simulink model "Simple_1MW_EVSE_SC_Study"  (R2024b)
settings: Solver=FixedStepDiscrete  StartTime=0.0  StopTime=10.0  FixedStep=1e-4  RelTol=1e-3
undefined symbols (not defined in the file): DiscIntNeverNeededParam
libraries: spsCurrentMeasurementLib x3, spsSeriesRLCBranchLib x3, spsVoltageMeasurementLib x3, spsIdealSwitchLib x3, spsControlledCurrentSourceLib x1, spsControlledVoltageSourceLib x1, spsDCVoltageSourceLib x1, spspowerguiLib x1
settings Model: NumberOfSteps=10000  SnapshotInterval=10000  Creator=SUDHAK1  LastModifiedBy=SUDHAK1

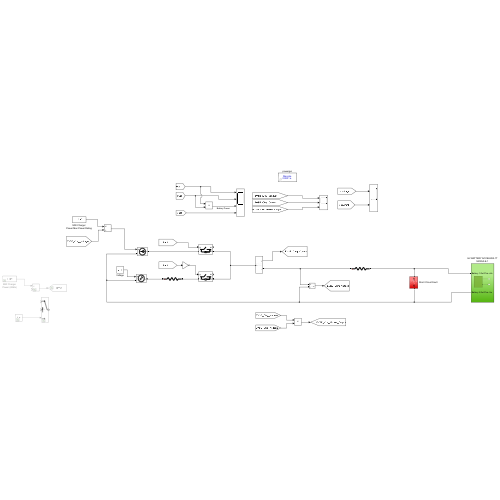
[thumbnail: Simulink's stored preview of the top-level diagram]
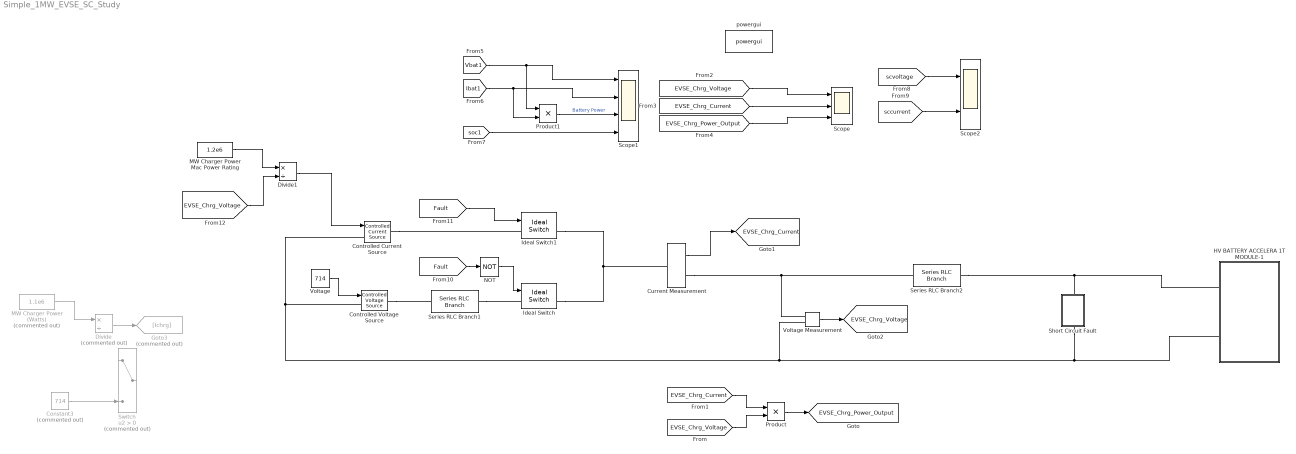
== system Simple_1MW_EVSE_SC_Study ==
  Constant3 : Constant  Commented=on  Value=714
  Controlled Current Source : spsControlledCurrentSourceLib/Controlled Current Source  Initialize=on  Source_Type=AC  Amplitude=0  Phase=0  Frequency=0  Measurements=None
  Controlled Voltage Source : spsControlledVoltageSourceLib/Controlled Voltage Source  Initialize=on  Source_Type=DC  Amplitude=0  Phase=0  Frequency=0  Measurements=None
  Current Measurement : spsCurrentMeasurementLib/Current Measurement  PhasorSimulation=off  OutputType=Complex  PSBequivalent=0
  Divide : Product  Commented=on  Inputs=*/
  Divide1 : Product  Inputs=*/
  Goto3 : Goto  Commented=on  GotoTag=Ichrg
  HV BATTERY ACCELERA 1T MODULE-1 : Subsystem
  Ideal Switch : spsIdealSwitchLib/Ideal Switch  Ron=1e-6  Lon=0  IC=0  Rs=1e5  Cs=inf  Measurements=on
  Ideal Switch1 : spsIdealSwitchLib/Ideal Switch  Ron=1e-6  Lon=0  IC=0  Rs=1e5  Cs=inf  Measurements=on
  MW Charger Power (Watts) : Constant  Commented=on  Value=1.1e6
  MW Charger Power Mac Power Rating : Constant  Value=1.2e6
  NOT : Logic  Operator=NOT  IconShape=distinctive  AllPortsSameDT=off  OutDataTypeStr=boolean
  Product : Product
  Product1 : Product
  Scope : Scope  NumInputPorts=3
  Scope1 : Scope  NumInputPorts=4
  Scope2 : Scope  NumInputPorts=2
  Series RLC Branch1 : spsSeriesRLCBranchLib/Series RLC Branch  LConnTagsString=__new0  RConnTagsString=__new0  BranchType=R  Resistance=(1000/1500)+0.3  Inductance=1e-3  SetiL0=off  InitialCurrent=0  Capacitance=1e-6  Setx0=off  InitialVoltage=0  Measurements=None
  Series RLC Branch2 : spsSeriesRLCBranchLib/Series RLC Branch  LConnTagsString=__new0  RConnTagsString=__new0  BranchType=R  Resistance=2e-3  Inductance=1e-3  SetiL0=off  InitialCurrent=0  Capacitance=1e-6  Setx0=off  InitialVoltage=0  Measurements=None
  Short Circuit Fault : Subsystem
      settings: PortSchema="{\"entries\":[{\"content\":{\"sides\":[{\"content\":{},\"type\":\"ConnectorPlacement.EquallySpacedRectSide\",\"uuid\":\"d1eece8f-50e0-4bd3-bd02-64a44f95c15f\"},{\"content\":{\"side\":\"RIGHT\"},\"type\":\"ConnectorPlacement.EquallySpacedRectSide\",\"uuid\":\"d3715762-f460-4a18-a379-b690b190937e\"},{\"content\":{\"connectorIds\":[\"LConn1\"],\"side\":\"TOP\"},\"type\":\"ConnectorPlacement.EquallySpacedRectSide\",\"uuid\":\"cdaaabb7-d644-4e36-8adb-959b7298db19\"},{\"content\":{\"connectorIds\":[\"RConn1\"],\"side\":\"BOTTOM\"},\"type\":\"ConnectorPlacement.EquallySpacedRectSide\",\"uuid\":\"a0244b95-e79a-4abc-836f-bd8cb9c3c8a7\"}]},\"type\":\"ConnectorPlacement.EquallySpacedConnector\",\"uuid\":\"f19808b0-397b-4bab-947c-d2711a911d87\"}],\"packageUris\":[\"http://schema.mathworks.com/mf0/Connector/R2020b\"],\"version\":\"1.0\"}"
  Switch : Switch  Commented=on  Criteria=u2 > Threshold  SaturateOnIntegerOverflow=off  InputSameDT=off
  Voltage : Constant  Value=714
  Voltage Measurement : spsVoltageMeasurementLib/Voltage Measurement  PhasorSimulation=off  OutputType=Complex  PSBequivalent=0
  powergui : spspowerguiLib/powergui  Priority=1  SimulationMode=Discrete  SampleTime=1e-4  frequency=60  Iterations=50  frequencyindice=0  Pbase=100e6  ErrMax=1e-4  UnitsV=kV  UnitsW=MW  buscounter=0  FunctionMessages=off  echomessages=off  EnableUseOfTLC=off  CurrentSourceSwitches=off  DisableSnubberDevices=off  DisableRonSwitches=off  DisableVfSwitches=off  DisplayEquations=off  AutomaticDiscreteSolvers=off  SolverType=Backward Euler  Interpol=off  ExternalGateDelay=off  methode=off  Ts=100  x0status=blocks  SPID=on  SwTol=0  HookPort=off  NonlinearTolerance=1e-4  nMaxIteration=100  ContinueOnMaxIteration=off  RestoreLinks=warning  ResistiveCurrentMeasurement=off  Frange=[0:2:500]  Ylog=off  Xlog=on  ShowGrid=off  save=off  variable=ZData  structure=0  ZoomFFT=off  StartTime=0.0  cycles=1  DisplayStyle=1  fundamental=60  FreqAxis=off  MaxFrequency=1000  frequencyindicesteady=1  RmsSteady=1  display=off
  tag scope: EVSE_Chrg_Current=global, EVSE_Chrg_Power_Output=global, EVSE_Chrg_Voltage=global
  wires:
  Product/1 -> [EVSE_Chrg_Power_Output]
  Current Measurement/1 -> [EVSE_Chrg_Current]
  Voltage Measurement/1 -> [EVSE_Chrg_Voltage]
  [EVSE_Chrg_Voltage] -> Product/2
  [EVSE_Chrg_Current] -> Product/1
  [EVSE_Chrg_Voltage] -> Scope/1
  [EVSE_Chrg_Current] -> Scope/2
  [EVSE_Chrg_Power_Output] -> Scope/3
  [Vbat1] -> Product1/1, Scope1/1
  [soc1] -> Scope1/4
  [Ibat1] -> Product1/2, Scope1/2
  Product1/1 -> Scope1/3  "Battery Power"
  [sccurrent] -> Scope2/2
  [scvoltage] -> Scope2/1
  Constant3/1 -> Switch/3
  Voltage/1 -> Controlled Voltage Source/1
  [Fault] -> NOT/1
  NOT/1 -> Ideal Switch/1
  [Fault] -> Ideal Switch1/1
  Divide/1 -> Goto3/1
  MW Charger Power (Watts)/1 -> Divide/1
  MW Charger Power Mac Power Rating/1 -> Divide1/1
  [EVSE_Chrg_Voltage] -> Divide1/2
  Divide1/1 -> Controlled Current Source/1
  connections:
  Current Measurement/RConn1 -- Series RLC Branch2/LConn1 -- Voltage Measurement/LConn1
  Controlled Voltage Source/RConn1 -- Series RLC Branch1/LConn1
  Short Circuit Fault/LConn1 -- Series RLC Branch2/RConn1 -- HV BATTERY ACCELERA 1T MODULE-1/RConn1
  Controlled Current Source/RConn1 -- Ideal Switch1/LConn1
  Ideal Switch/RConn1 -- Ideal Switch1/RConn1 -- Current Measurement/LConn1
  Series RLC Branch1/RConn1 -- Ideal Switch/LConn1
  Short Circuit Fault/RConn1 -- Voltage Measurement/LConn2 -- Controlled Voltage Source/LConn1 -- Controlled Current Source/LConn1 -- HV BATTERY ACCELERA 1T MODULE-1/RConn2

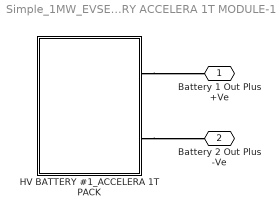
== system Simple_1MW_EVSE_SC_Study/HV BATTERY ACCELERA 1T MODULE-1 ==
  HV BATTERY #1_ACCELERA 1T PACK : Subsystem
  Battery 1 Out Plus +Ve : PMIOPort  Side=Right
  Battery 2 Out Plus -Ve : PMIOPort  Port=2  Side=Right
  connections:
  HV BATTERY #1_ACCELERA 1T PACK/RConn1 -- Battery 1 Out Plus +Ve/RConn1
  HV BATTERY #1_ACCELERA 1T PACK/RConn2 -- Battery 2 Out Plus -Ve/RConn1

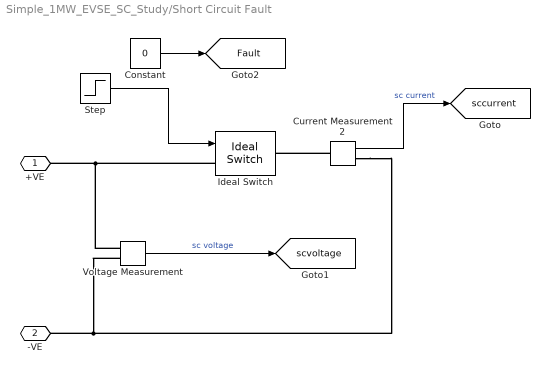
== system Simple_1MW_EVSE_SC_Study/Short Circuit Fault ==
  Constant : Constant  Value=0
  Current Measurement2 : spsCurrentMeasurementLib/Current Measurement  PhasorSimulation=off  OutputType=Complex  PSBequivalent=0
  Ideal Switch : spsIdealSwitchLib/Ideal Switch  Ron=5e-3  Lon=0  IC=0  Rs=1e5  Cs=inf  Measurements=off
  Step : Step  Time=2  SampleTime=0
  Voltage Measurement : spsVoltageMeasurementLib/Voltage Measurement  PhasorSimulation=off  OutputType=Complex  PSBequivalent=0
  +VE : PMIOPort  Side=Left
  -VE : PMIOPort  Port=2  Side=Right
  tag scope: Fault=global, sccurrent=global, scvoltage=global
  wires:
  Step/1 -> Ideal Switch/1
  Current Measurement2/1 -> [sccurrent]  "sc current"
  Voltage Measurement/1 -> [scvoltage]  "sc voltage"
  Constant/1 -> [Fault]
  connections:
  Current Measurement2/RConn1 -- Voltage Measurement/LConn2 -- -VE/RConn1
  Ideal Switch/LConn1 -- Voltage Measurement/LConn1 -- +VE/RConn1
  Current Measurement2/LConn1 -- Ideal Switch/RConn1

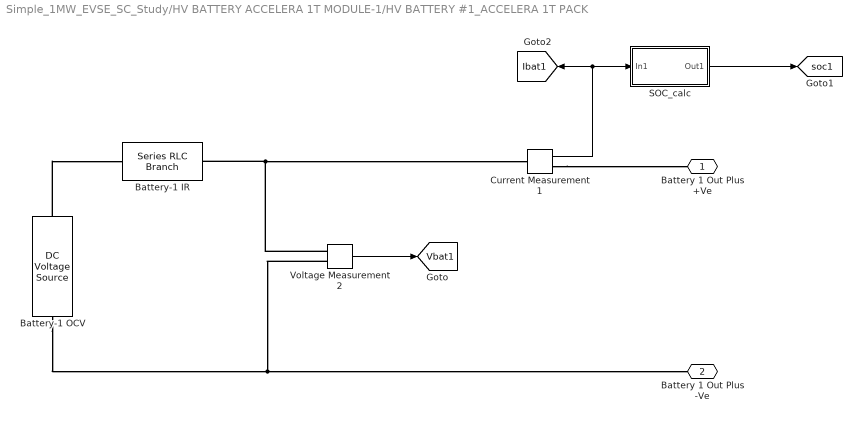
== system Simple_1MW_EVSE_SC_Study/HV BATTERY ACCELERA 1T MODULE-1/HV BATTERY #1_ACCELERA 1T PACK ==
  Battery-1 IR : spsSeriesRLCBranchLib/Series RLC Branch  LConnTagsString=__new0  RConnTagsString=__new0  BranchType=R  Resistance=0.003691539  Inductance=1e-3  SetiL0=off  InitialCurrent=0  Capacitance=1e-6  Setx0=off  InitialVoltage=0  Measurements=None
  Battery-1 OCV : spsDCVoltageSourceLib/DC Voltage Source  Amplitude=649.32  Measurements=None
  Current Measurement1 : spsCurrentMeasurementLib/Current Measurement  PhasorSimulation=off  OutputType=Complex  PSBequivalent=0
  SOC_calc : Subsystem
  Voltage Measurement2 : spsVoltageMeasurementLib/Voltage Measurement  PhasorSimulation=off  OutputType=Complex  PSBequivalent=0
  Battery 1 Out Plus +Ve : PMIOPort  Side=Right
  Battery 1 Out Plus -Ve : PMIOPort  Port=2  Side=Right
  tag scope: Ibat1=global, Vbat1=global, soc1=global
  wires:
  Voltage Measurement2/1 -> [Vbat1]
  SOC_calc/1(Out1) -> [soc1]
  Current Measurement1/1 -> [Ibat1], SOC_calc/1(In1)
  connections:
  Voltage Measurement2/LConn2 -- Battery-1 OCV/LConn1 -- Battery 1 Out Plus -Ve/RConn1
  Voltage Measurement2/LConn1 -- Current Measurement1/LConn1 -- Battery-1 IR/RConn1
  Current Measurement1/RConn1 -- Battery 1 Out Plus +Ve/RConn1
  Battery-1 OCV/RConn1 -- Battery-1 IR/LConn1

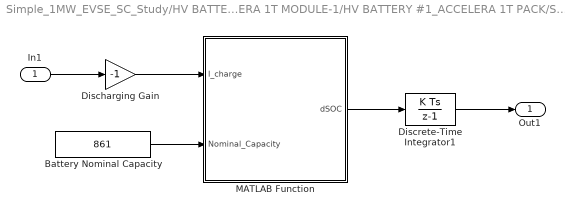
== system Simple_1MW_EVSE_SC_Study/HV BATTERY ACCELERA 1T MODULE-1/HV BATTERY #1_ACCELERA 1T PACK/SOC_calc ==
  In1 : Inport
  Battery Nominal Capacity : Constant  Value=861
  Discharging Gain : Gain  Gain=-1
  Discrete-Time Integrator1 : DiscreteIntegrator  InitialCondition=5  SampleTime=-1  LimitOutput=on  UpperSaturationLimit=100  LowerSaturationLimit=0  ICPrevOutput=DiscIntNeverNeededParam  ICPrevScaledInput=DiscIntNeverNeededParam
  MATLAB Function : MATLAB Function  TreatAsAtomicUnit=on
  Out1 : Outport
  wires:
  In1/1 -> Discharging Gain/1
  Discrete-Time Integrator1/1 -> Out1/1
  MATLAB Function/1(dSOC) -> Discrete-Time Integrator1/1
  Discharging Gain/1 -> MATLAB Function/1(I_charge)
  Battery Nominal Capacity/1 -> MATLAB Function/2(Nominal_Capacity)

== matlab function Simple_1MW_EVSE_SC_Study/HV BATTERY ACCELERA 1T MODULE-1/HV BATTERY #1_ACCELERA 1T PACK/SOC_calc/MATLAB Function ==
  data: I_charge input; dSOC output; Nominal_Capacity input
function dSOC = calculate_SOC_Decrement(I_charge,Nominal_Capacity)
% Function to calculate SOC increment for a single battery
% Input:
%   I_charge - Charging current for the battery (A)
% Output:
%   dSOC - Incremental SOC (%)

% Battery parameters
Q_capacity = Nominal_Capacity;    % Battery capacity in Ah
eta = 1;          % Charging efficiency

% Calculate the SOC increment
dSOC = (eta * I_charge) / Q_capacity * 100 / 3600; % SOC change per second
end
